simulink model "ARDroneReplay_V2_backup_2026-11-12"  (R2025b)
settings: Solver=ode1  StartTime=0.0  StopTime=45.145  FixedStep=sampleTime  RelTol=1e-3  EnableMultiTasking=on
values from neighbouring files (symbols this model uses):
  sampleTime = 1/200    (= 0.005)    [setupReplay.m]
undefined symbols (not defined in the file or in its folder): A, B, C, KALMAN_GAIN
libraries: ARBlocks x2
settings Model: ExtModeTrigDuration=100000  Creator=Paul  LastModifiedBy=caio
settings SolverCC: AlgebraicLoopSolver=TrustRegion
settings DataIOCC: LimitDataPoints=on  SaveFormat=Array  SignalLoggingSaveFormat=ModelDataLogs  ReturnWorkspaceOutputs=off  TimeSaveName=time
settings OptimizationCC: ExpressionDepthLimit=2147483647.0  InitFltsAndDblsToZero=on
settings DebuggingCC: UnderspecifiedInitializationDetection=Classic  MergeDetectMultiDrivingBlocksExec=none  SolverPrmCheckMsg=warning  FcnCallInpInsideContextMsg=warning  UnconnectedInputMsg=warning  UnconnectedOutputMsg=warning  UnconnectedLineMsg=warning  StateNameClashWarn=warning  SFUnexpectedBacktrackingDiag=warning  SFNoUnconditionalDefaultTransitionDiag=warning  SFExecutionAtInitializationDiag=none  ArithmeticOperatorsInVariantConditions=warning
settings HardwareCC: ProdBitPerLong=64.0  ProdHWDeviceType=Intel->x86-64 (Linux 64)
settings ModelReferenceCC: EnableRefExpFcnMdlSchedulingChecks=on  PropagateSignalLabelsOutOfModel=off
settings SFSimCC: SimUseLocalCustomCode=off  CustomCodeUndefinedFunction=UseInterfaceOnly
settings RTWCC: SystemTargetFile=sldrt.tlc  TemplateMakefile=sldrt.tmf  RTWUseLocalCustomCode=off  RTWCompilerOptimization=on  GPUComputeCapability=3.5  Description=Simulink Desktop Real-Time
settings CodeAppCC: MaxIdLength=95.0  StateflowObjectComments=on
settings SimulinkDesktopRealTimeCC: ExtModeTransport=0.0  ExtModeStaticAllocSize=1000000.0  TargetLibSuffix=_sldrt.a  TargetPreCompLibLocation=/home/caio/.local/share/MATLAB/R2025b/toolbox/sldrt/lib/glnxa64  TargetLangStandard=C89/C90 (ANSI)  MultiwordLength=2048.0  DynamicStringBufferSize=256.0  ParMdlRefBuildCompliant=on  PreserveMATLABNamespacesInGeneratedCode=on  SubcomponentCodeInterfacePackaging=Reusable function  SupportVariableSizeSignals=off
settings ConfigComp: CovMetricSettings=dw  CovSaveCumulativeToWorkspaceVar=on  CovSaveSingleToWorkspaceVar=on  CovExternalEMLEnable=off

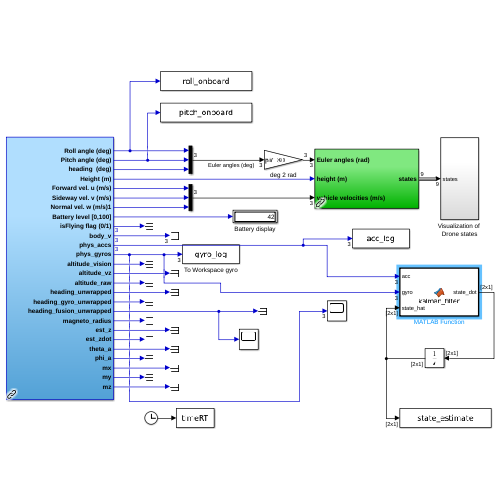
[thumbnail: Simulink's stored preview of the top-level diagram]
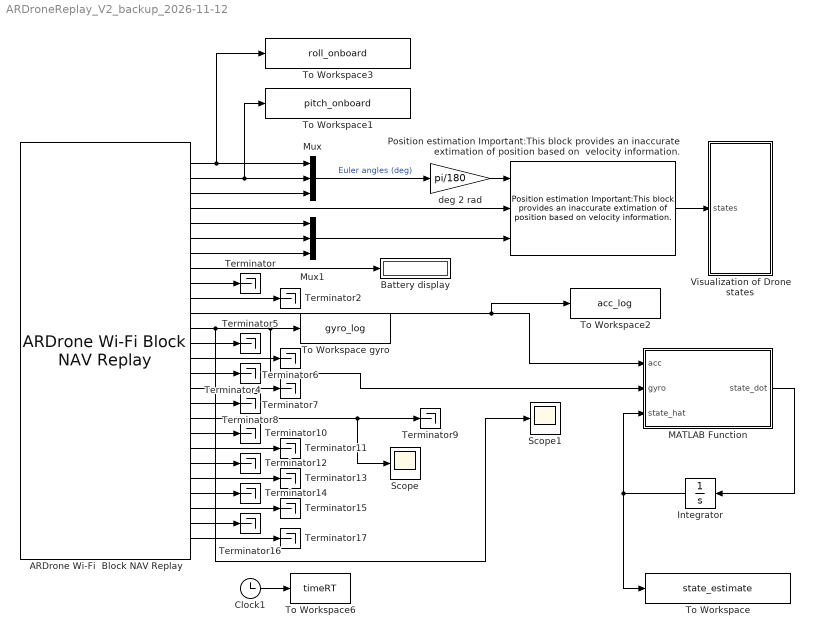
== system ARDroneReplay_V2_backup_2026-11-12 ==
  ARDrone Wi-Fi  Block NAV Replay : ARBlocks/ARDrone Wi-Fi  Block NAV Replay  SystemSampleTime=-1  VariantActivationTime=update diagram  EmptyChoice=off  PassThrough=off  PassThroughVariantControl=(default)  EmptyChoiceVariantControl=(default)  AllowFlexibleInterface=on  Latency=0  AutoFrameSizeCalculation=off
  Battery display : Display
  Clock1 : Clock
  Integrator : Integrator  InitialCondition=zeros(size(A,1), 1)
  MATLAB Function : MATLAB Function  TreatAsAtomicUnit=on
  Mux : Mux  Inputs=3
  Mux1 : Mux  Inputs=3
  "Position estimation Important:This block provides an inaccurate extimation of position based on  velocity information. " : ARBlocks/Position estimation Important:This block provides an  inaccurate extimation of position  based on  velocity information.   SystemSampleTime=-1  VariantActivationTime=update diagram  EmptyChoice=off  PassThrough=off  PassThroughVariantControl=(default)  EmptyChoiceVariantControl=(default)  AllowFlexibleInterface=on  Latency=0  AutoFrameSizeCalculation=off
  Scope : Scope
      settings: ActiveDisplayYMinimum=-0.58202  ActiveDisplayYMaximum=1.32261
  Scope1 : Scope
      settings: ActiveDisplayYMinimum=-0.28836918249726295  ActiveDisplayYMaximum=0.25480991974473
  Terminator{,2,4..17} (16 alike) : Terminator
  To Workspace : ToWorkspace  VariableName=state_estimate  SaveFormat=Structure With Time  SampleTime=-1
  To Workspace gyro : ToWorkspace  VariableName=gyro_log  SaveFormat=Structure With Time  SampleTime=-1
  To Workspace1 : ToWorkspace  VariableName=pitch_onboard  SaveFormat=Structure With Time  SampleTime=-1
  To Workspace2 : ToWorkspace  VariableName=acc_log  SaveFormat=Structure With Time  SampleTime=-1
  To Workspace3 : ToWorkspace  VariableName=roll_onboard  SaveFormat=Structure With Time  SampleTime=-1
  To Workspace6 : ToWorkspace  VariableName=timeRT  SampleTime=sampleTime
  Visualization of Drone states : Subsystem
  deg 2 rad : Gain  Gain=pi/180
  wires:
  ARDrone Wi-Fi  Block NAV Replay/1 -> To Workspace3/1, Mux/1
  ARDrone Wi-Fi  Block NAV Replay/2 -> To Workspace1/1, Mux/2
  ARDrone Wi-Fi  Block NAV Replay/5 -> Mux1/1
  ARDrone Wi-Fi  Block NAV Replay/6 -> Mux1/2
  ARDrone Wi-Fi  Block NAV Replay/7 -> Mux1/3
  Mux/1 -> deg 2 rad/1  "Euler angles (deg)"
  ARDrone Wi-Fi  Block NAV Replay/8 -> Battery display/1
  "Position estimation Important:This block provides an inaccurate extimation of position based on  velocity information. "/1 -> Visualization of Drone states/1(states)
  deg 2 rad/1 -> "Position estimation Important:This block provides an inaccurate extimation of position based on  velocity information. "/1
  ARDrone Wi-Fi  Block NAV Replay/4 -> "Position estimation Important:This block provides an inaccurate extimation of position based on  velocity information. "/2
  Mux1/1 -> "Position estimation Important:This block provides an inaccurate extimation of position based on  velocity information. "/3
  ARDrone Wi-Fi  Block NAV Replay/3 -> Mux/3
  ARDrone Wi-Fi  Block NAV Replay/9 -> Terminator/1
  Clock1/1 -> To Workspace6/1
  ARDrone Wi-Fi  Block NAV Replay/15 -> Terminator4/1
  ARDrone Wi-Fi  Block NAV Replay/10 -> Terminator2/1
  ARDrone Wi-Fi  Block NAV Replay/13 -> Terminator5/1
  ARDrone Wi-Fi  Block NAV Replay/14 -> Terminator6/1
  ARDrone Wi-Fi  Block NAV Replay/17 -> Terminator8/1
  ARDrone Wi-Fi  Block NAV Replay/16 -> Terminator7/1
  ARDrone Wi-Fi  Block NAV Replay/19 -> Terminator10/1
  ARDrone Wi-Fi  Block NAV Replay/18 -> Scope/1, Terminator9/1
  ARDrone Wi-Fi  Block NAV Replay/21 -> Terminator12/1
  ARDrone Wi-Fi  Block NAV Replay/20 -> Terminator11/1
  ARDrone Wi-Fi  Block NAV Replay/23 -> Terminator14/1
  ARDrone Wi-Fi  Block NAV Replay/22 -> Terminator13/1
  ARDrone Wi-Fi  Block NAV Replay/25 -> Terminator16/1
  ARDrone Wi-Fi  Block NAV Replay/24 -> Terminator15/1
  ARDrone Wi-Fi  Block NAV Replay/26 -> Terminator17/1
  ARDrone Wi-Fi  Block NAV Replay/11 -> To Workspace2/1, MATLAB Function/1(acc)
  MATLAB Function/1(state_dot) -> Integrator/1
  Integrator/1 -> To Workspace/1, MATLAB Function/3(state_hat)
  ARDrone Wi-Fi  Block NAV Replay/12 -> To Workspace gyro/1, MATLAB Function/2(gyro), Scope1/1

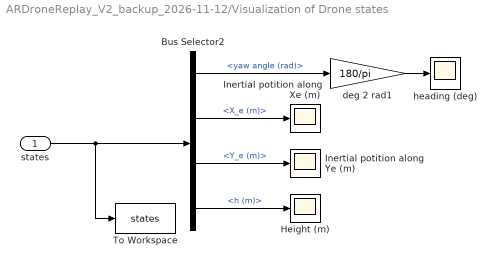
== system ARDroneReplay_V2_backup_2026-11-12/Visualization of Drone states ==
  states : Inport
  Bus Selector2 : BusSelector  OutputSignals=yaw angle (rad),X_e (m),Y_e (m),h (m)
  Height (m) : Scope
      settings: ActiveDisplayYMinimum=-0.15212  ActiveDisplayYMaximum=1.36913  DataLoggingMaxPoints=500000  DataLoggingVariableName=ScopeData5
  Inertial potition along Xe (m) : Scope
      settings: ActiveDisplayYMinimum=-0.49449  ActiveDisplayYMaximum=0.46559  DataLoggingMaxPoints=500000  DataLoggingVariableName=ScopeData3
  Inertial potition along Ye (m) : Scope
      settings: ActiveDisplayYMinimum=-0.28577  ActiveDisplayYMaximum=0.69906  DataLoggingMaxPoints=500000  DataLoggingVariableName=ScopeData4
  To Workspace : ToWorkspace  VariableName=states  SaveFormat=Structure With Time  SampleTime=-1
  deg 2 rad1 : Gain  Gain=180/pi
  heading (deg) : Scope
      settings: ActiveDisplayYMinimum=-139.82962  ActiveDisplayYMaximum=15.53662  DataLoggingMaxPoints=500000  DataLoggingVariableName=ScopeData2
  wires:
  states/1 -> To Workspace/1, Bus Selector2/1
  Bus Selector2/1 -> deg 2 rad1/1  "<yaw angle (rad)>"
  Bus Selector2/2 -> Inertial potition along Xe (m)/1  "<X_e (m)>"
  Bus Selector2/3 -> Inertial potition along Ye (m)/1  "<Y_e (m)>"
  Bus Selector2/4 -> Height (m)/1  "<h (m)>"
  deg 2 rad1/1 -> heading (deg)/1

== matlab function ARDroneReplay_V2_backup_2026-11-12/MATLAB Function ==
  data: acc input; gyro input; state_dot output; state_hat input; A parameter; B parameter; C parameter; KALMAN_GAIN parameter
function state_dot = kalman_filter(acc, gyro, state_hat, A, B, C, KALMAN_GAIN)
    u = [gyro(1); gyro(2)] * pi/180;
    y = [atan2(-acc(2), -acc(3)); atan2(acc(1), sqrt(acc(2)^2 + acc(3)^2))];
    state_dot = A * state_hat + B * u + KALMAN_GAIN * (y - C * state_hat);
end
